simulink model "HW6"  (R2023b)
settings: Solver=FixedStepAuto  StartTime=0.0  StopTime=20  FixedStep=0.001  RelTol=1e-3
settings Model: Creator=ArshiaGosh  LastModifiedBy=ArshiaGosh

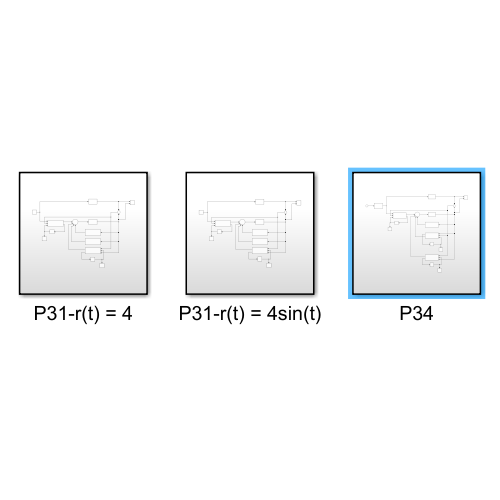
[thumbnail: Simulink's stored preview of the top-level diagram]
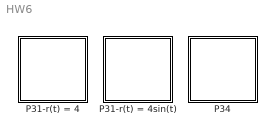
== system HW6 ==
  P31-r(t) = 4 : Subsystem
  P31-r(t) = 4sin(t) : Subsystem
  P34 : Subsystem

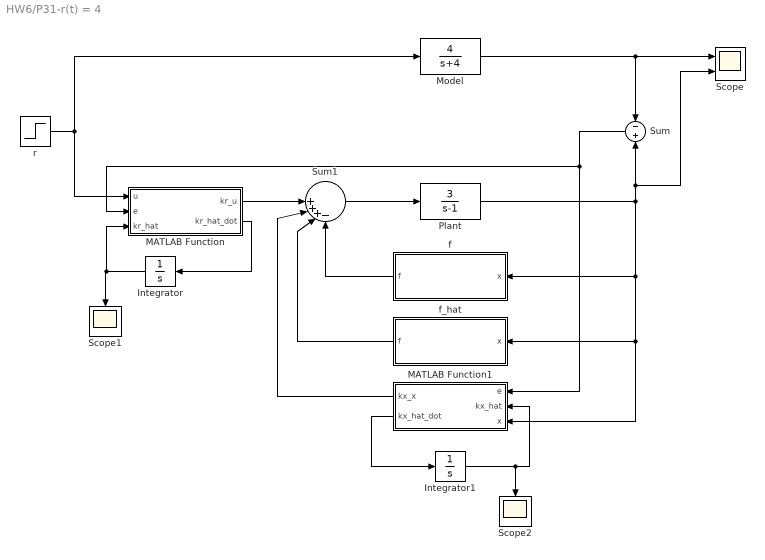
== system HW6/P31-r(t) = 4 ==
  Integrator : Integrator
  Integrator1 : Integrator
  MATLAB Function : MATLAB Function  TreatAsAtomicUnit=on
  MATLAB Function1 : MATLAB Function  TreatAsAtomicUnit=on
  Model : TransferFcn  Numerator=[4]  Denominator=[1 4]
  Plant : TransferFcn  Numerator=[3]  Denominator=[1 -1]
  Scope : Scope  NumInputPorts=2
  Scope1 : Scope
  Scope2 : Scope
  Sum : Sum  Inputs=-|+
  Sum1 : Sum  Inputs=|||+++-
  f : MATLAB Function  TreatAsAtomicUnit=on
  f_hat : MATLAB Function  TreatAsAtomicUnit=on
  r : Step  Time=0  After=4  SampleTime=0
  wires:
  MATLAB Function/1(kr_u) -> Sum1/1
  MATLAB Function1/1(kx_x) -> Sum1/2
  f_hat/1(f) -> Sum1/3
  Integrator/1 -> Scope1/1, MATLAB Function/3(kr_hat)
  Integrator1/1 -> MATLAB Function1/2(kx_hat), Scope2/1
  MATLAB Function1/2(kx_hat_dot) -> Integrator1/1
  MATLAB Function/2(kr_hat_dot) -> Integrator/1
  Sum1/1 -> Plant/1
  Model/1 -> Scope/1, Sum/1
  Sum/1 -> MATLAB Function/2(e), MATLAB Function1/1(e)
  r/1 -> MATLAB Function/1(u), Model/1
  f/1(f) -> Sum1/4
  Plant/1 -> MATLAB Function1/3(x), f_hat/1(x), f/1(x), Scope/2, Sum/2

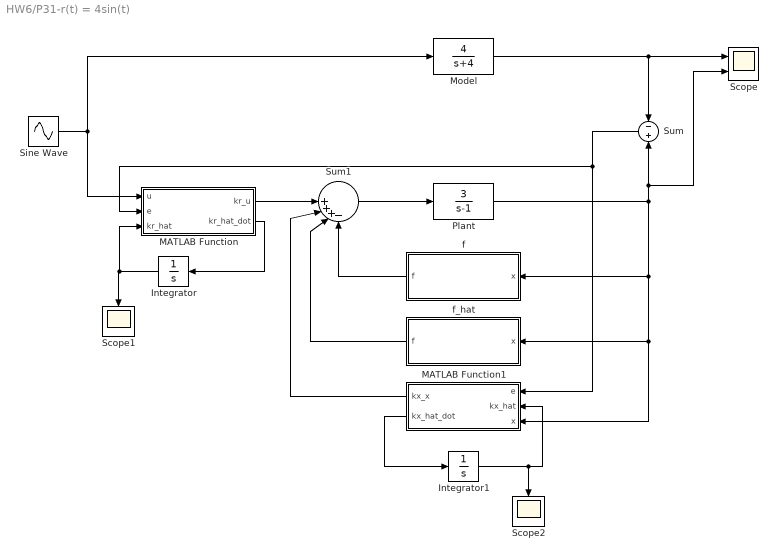
== system HW6/P31-r(t) = 4sin(t) ==
  Integrator : Integrator
  Integrator1 : Integrator
  MATLAB Function : MATLAB Function  TreatAsAtomicUnit=on
  MATLAB Function1 : MATLAB Function  TreatAsAtomicUnit=on
  Model : TransferFcn  Numerator=[4]  Denominator=[1 4]
  Plant : TransferFcn  Numerator=[3]  Denominator=[1 -1]
  Scope : Scope  NumInputPorts=2
  Scope1 : Scope
  Scope2 : Scope
  Sine Wave : Sin  Amplitude=4  Frequency=3  SampleTime=0
  Sum : Sum  Inputs=-|+
  Sum1 : Sum  Inputs=|||+++-
  f : MATLAB Function  TreatAsAtomicUnit=on
  f_hat : MATLAB Function  TreatAsAtomicUnit=on
  wires:
  Plant/1 -> Sum/2, Scope/2, f/1(x), f_hat/1(x), MATLAB Function1/3(x)
  f/1(f) -> Sum1/4
  Sine Wave/1 -> Model/1, MATLAB Function/1(u)
  Sum/1 -> MATLAB Function1/1(e), MATLAB Function/2(e)
  Model/1 -> Sum/1, Scope/1
  Sum1/1 -> Plant/1
  MATLAB Function/2(kr_hat_dot) -> Integrator/1
  MATLAB Function1/2(kx_hat_dot) -> Integrator1/1
  Integrator1/1 -> Scope2/1, MATLAB Function1/2(kx_hat)
  Integrator/1 -> MATLAB Function/3(kr_hat), Scope1/1
  f_hat/1(f) -> Sum1/3
  MATLAB Function1/1(kx_x) -> Sum1/2
  MATLAB Function/1(kr_u) -> Sum1/1

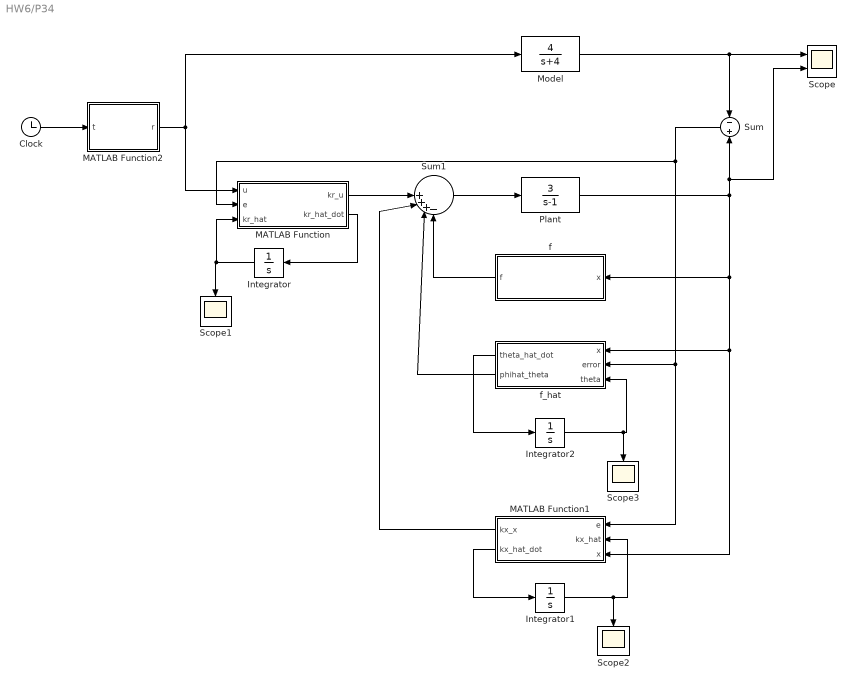
== system HW6/P34 ==
  Clock : Clock
  Integrator : Integrator
  Integrator1 : Integrator
  Integrator2 : Integrator  InitialCondition=[0;0;0;0]
  MATLAB Function : MATLAB Function  TreatAsAtomicUnit=on
  MATLAB Function1 : MATLAB Function  TreatAsAtomicUnit=on
  MATLAB Function2 : MATLAB Function  TreatAsAtomicUnit=on
  Model : TransferFcn  Numerator=[4]  Denominator=[1 4]
  Plant : TransferFcn  Numerator=[3]  Denominator=[1 -1]
  Scope : Scope  NumInputPorts=2
  Scope1 : Scope
  Scope2 : Scope
  Scope3 : Scope
  Sum : Sum  Inputs=-|+
  Sum1 : Sum  Inputs=|||+++-
  f : MATLAB Function  TreatAsAtomicUnit=on
  f_hat : MATLAB Function  TreatAsAtomicUnit=on
  wires:
  Plant/1 -> Sum/2, Scope/2, f/1(x), MATLAB Function1/3(x), f_hat/1(x)
  f/1(f) -> Sum1/4
  MATLAB Function2/1(r) -> Model/1, MATLAB Function/1(u)
  Sum/1 -> MATLAB Function1/1(e), f_hat/2(error), MATLAB Function/2(e)
  Model/1 -> Sum/1, Scope/1
  Sum1/1 -> Plant/1
  MATLAB Function/2(kr_hat_dot) -> Integrator/1
  MATLAB Function1/2(kx_hat_dot) -> Integrator1/1
  Integrator1/1 -> Scope2/1, MATLAB Function1/2(kx_hat)
  Integrator/1 -> MATLAB Function/3(kr_hat), Scope1/1
  MATLAB Function1/1(kx_x) -> Sum1/2
  MATLAB Function/1(kr_u) -> Sum1/1
  Clock/1 -> MATLAB Function2/1(t)
  Integrator2/1 -> f_hat/3(theta), Scope3/1
  f_hat/1(theta_hat_dot) -> Integrator2/1
  f_hat/2(phihat_theta) -> Sum1/3

== matlab function HW6/P34/f ==
  data: f output; x input
function f  = fcn(x)
phi_x = [x^3; exp(-((x+0.5)^2) * 10); exp(-((x-0.5)^2) * 10); sin(2*x)];
theta = [0.01; -1; 1 ; 0.5];
f = phi_x'*theta;
end

== matlab function HW6/P34/f_hat ==
  data: theta_hat_dot output size=4; x input; error input; theta input; phihat_theta output
function [theta_hat_dot, phihat_theta] = fcn(x,error,theta)
phi_x = [x^3; exp(-((x+0.5)^2) * 10); exp(-((x-0.5)^2) * 10); sin(2*x)];
theta_hat_dot = -2.*phi_x.*error;
phihat_theta = theta' * phi_x;
end

== matlab function HW6/P34/MATLAB Function2 ==
  data: t input; r output
function r = fcn(t)
r = sin(3*t) + sin(3*t/2) + sin(3*t/4) + sin(3*t/8);
end

== matlab function HW6/P31-r(t) = 4/f ==
  data: f output; x input
function f  = fcn(x)
f = 0;
end

== matlab function HW6/P31-r(t) = 4/MATLAB Function ==
  data: u input; kr_u output; e input; kr_hat input; kr_hat_dot output
function [kr_u, kr_hat_dot] = fcn(u, e, kr_hat)
kr_u = kr_hat * u;
kr_hat_dot = -2*u*e;
end

== matlab function HW6/P31-r(t) = 4/f_hat ==
  data: f output; x input
function f  = fcn(x)
f = 0;
end

== matlab function HW6/P31-r(t) = 4/MATLAB Function1 ==
  data: e input; kx_hat input; kx_x output; kx_hat_dot output; x input
function [kx_x, kx_hat_dot] = fcn(e, kx_hat,x)
kx_x = kx_hat * x;
kx_hat_dot = -2*x*e;
end

== matlab function HW6/P31-r(t) = 4sin(t)/MATLAB Function ==
  data: u input; kr_u output; e input; kr_hat input; kr_hat_dot output
function [kr_u, kr_hat_dot] = fcn(u, e, kr_hat)
kr_u = kr_hat * u;
kr_hat_dot = -2*u*e;
end

== matlab function HW6/P31-r(t) = 4sin(t)/MATLAB Function1 ==
  data: e input; kx_hat input; kx_x output; kx_hat_dot output; x input
function [kx_x, kx_hat_dot] = fcn(e, kx_hat,x)
kx_x = kx_hat * x;
kx_hat_dot = -2*x*e;
end

== matlab function HW6/P31-r(t) = 4sin(t)/f ==
  data: f output; x input
function f  = fcn(x)
f = 0;
end

== matlab function HW6/P31-r(t) = 4sin(t)/f_hat ==
  data: f output; x input
function f  = fcn(x)
f = 0;
end

== matlab function HW6/P34/MATLAB Function ==
  data: u input; kr_u output; e input; kr_hat input; kr_hat_dot output
function [kr_u, kr_hat_dot] = fcn(u, e, kr_hat)
kr_u = kr_hat * u;
kr_hat_dot = -2*u*e;
end

== matlab function HW6/P34/MATLAB Function1 ==
  data: e input; kx_hat input; kx_x output; kx_hat_dot output; x input
function [kx_x, kx_hat_dot] = fcn(e, kx_hat,x)
kx_x = kx_hat * x;
kx_hat_dot = -2*x*e;
end
